simulink model "My_gfm_battery_sil_1"  (R2018b)
settings: Solver=ode23t  StartTime=0.0  StopTime=30  MaxStep=1e-4  RelTol=1e-3
PreLoadFcn:
  | modelDir = fileparts(get_param(bdroot,'FileName'));
  | 
  | load_system(fullfile(modelDir,'controls_element_lib.slx'));
  | load_system(fullfile(modelDir,'test_sequence_lib.slx'));
InitFcn:
  | close all;
  | clear all;
  | clc;
  | 
  | % frequency nominals
  | F_NOM = 60;
  | W_NOM = 2 * pi * F_NOM;
  | 
  | % base values relative to inverter
  | % --------------------------------
  | VLL_INV_NOM = 480;
  | P_INV_NOM = 1e6;
  | Q_INV_NOM = 0.5e6;
  | S_INV_NOM = sqrt(P_INV_NOM^2 + Q_INV_NOM^2);
  | 
  | I_INV_BASE = S_INV_NOM/(sqrt(3)*VLL_INV_NOM);
  | Z_INV_BASE = VLL_INV_NOM^2/S_INV_NOM;
  | L_INV_BASE = Z_INV_BASE / W_NOM;
  | C_INV_BASE = 1 / (Z_INV_BASE * W_NOM);
  | 
  | % nominal ratings for power system model
  | % --------------------------------------
  | INVERTER_COUNT = 100;
  | 
  | VLV_NOM = VLL_INV_NOM;
  | VMV_NOM = 35e3;
  | VHV_NOM = 230e3;
  | S_PLANT = INVERTER_COUNT * S_INV_NOM;
  | 
  | N_GSU = VHV_NOM/VMV_NOM;
  | N_MVT = VMV_NOM/VLV_NOM;
  | 
  | I_LV_BASE = S_PLANT/(sqrt(3)*VLV_NOM);
  | I_MV_BASE = S_PLANT/(sqrt(3)*VMV_NOM);
  | I_HV_BASE = S_PLANT/(sqrt(3)*VHV_NOM);
  | 
  | Z_LV_BASE = VLV_NOM^2/S_PLANT;
  | Z_MV_BASE = VMV_NOM^2/S_PLANT;
  | Z_HV_BASE = VHV_NOM^2/S_PLANT;
  | 
  | L_LV_BASE = Z_LV_BASE / W_NOM;
  | L_MV_BASE = Z_MV_BASE / W_NOM;
  | L_HV_BASE = Z_HV_BASE / W_NOM;
  | C_LV_BASE = 1 / (Z_LV_BASE * W_NOM);
  | C_MV_BASE = 1 / (Z_MV_BASE * W_NOM);
  | C_HV_BASE = 1 / (Z_HV_BASE * W_NOM);
undefined symbols (not defined in the file): j
libraries: simulink x38, test_sequence_lib x10, controls_element_lib x9
(part 1 of 5)
settings Model: SimulationMode=accelerator  Creator=HussamAlatrash  LastModifiedBy=ahhei
settings DataIOCC: ReturnWorkspaceOutputs=on
settings OptimizationCC: EfficientMapNaN2IntZero=off
settings DebuggingCC: UnconnectedInputMsg=none  UnconnectedOutputMsg=none  UnconnectedLineMsg=none
settings HardwareCC: TargetBitPerPointer=64  TargetBitPerSizeT=64  TargetBitPerPtrDiffT=64  TargetLongLongMode=on  TargetIntDivRoundTo=Zero  TargetEndianess=LittleEndian  TargetWordSize=64  TargetHWDeviceType=MATLAB Host  ProdEqTarget=off
settings ModelReferenceCC: EnableRefExpFcnMdlSchedulingChecks=off
settings CodeAppCC: MaxIdLength=128
settings GRTTargetCC: TargetLangStandard=C89/C90 (ANSI)  CombineOutputUpdateFcns=off  GRTInterface=on

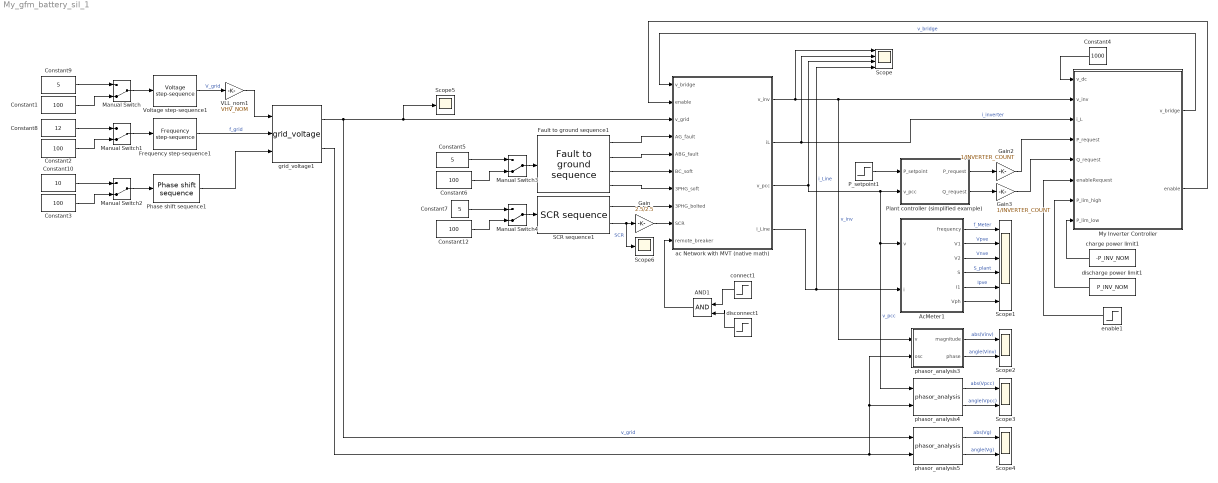
== system My_gfm_battery_sil_1 ==
  AND1 : Logic  IconShape=distinctive  AllPortsSameDT=off  OutDataTypeStr=boolean
  AcMeter1 : Subsystem  AncestorBlock=test_sequence_lib/AcMeter  mask{VllRated=VHV_NOM}
      mask prompts: VllRated "Rated line voltage"
  Constant{1..3,6,12} (5 alike) : Constant  Value=100
  Constant10 : Constant  Value=10
  Constant4 : Constant  Value=1000
  Constant5 : Constant  Value=5
  Constant7 : Constant  Value=5
  Constant8 : Constant  Value=12
  Constant9 : Constant  Value=5
  Fault to ground sequence1 : test_sequence_lib/Fault to ground sequence  SystemSampleTime=-1
  Frequency step-sequence1 : test_sequence_lib/Frequency step-sequence  SystemSampleTime=-1
  Gain : Gain  Gain=2.5/2.5
  Gain2 : Gain  Gain=1/INVERTER_COUNT
  Gain3 : Gain  Gain=1/INVERTER_COUNT
  Manual Switch{,1..4} (5 alike) : ManualSwitch  CurrentSetting=0
  "My Inverter Controller " : Subsystem
  P_setpoint1 : Step  Time=4  After=S_PLANT*0.9  SampleTime=0
  Phase shift sequence1 : test_sequence_lib/Phase shift sequence  SystemSampleTime=-1
  Plant controller (simplified example) : Subsystem  AncestorBlock=controls_element_lib/Battery plant controller
  SCR sequence1 : test_sequence_lib/SCR sequence  SystemSampleTime=-1
  Scope : Scope  NumInputPorts=4
  Scope1 : Scope  NumInputPorts=6
  Scope2 : Scope  NumInputPorts=2
  Scope3 : Scope  NumInputPorts=2
  Scope4 : Scope  NumInputPorts=2
  Scope5 : Scope
  Scope6 : Scope
  VLL_nom1 : Gain  Gain=VHV_NOM
  Voltage step-sequence1 : test_sequence_lib/Voltage step-sequence  SystemSampleTime=-1
  ac Network with MVT (native math) : Subsystem  AncestorBlock=test_sequence_lib/ac Network with MVT (native math)
  charge power limit1 : Constant  Value=-P_INV_NOM
  connect1 : Step  Time=0  SampleTime=0
  discharge power limit1 : Constant  Value=P_INV_NOM
  disconnect1 : Step  Time=100  Before=1  After=0  SampleTime=0
  enable1 : Step  Time=0.5  SampleTime=0
  grid_voltage1 : test_sequence_lib/grid_voltage  SystemSampleTime=-1
  phasor_analysis3 : Subsystem  AncestorBlock=test_sequence_lib/phasor_analysis
  phasor_analysis4 : test_sequence_lib/phasor_analysis  SystemSampleTime=-1
  phasor_analysis5 : test_sequence_lib/phasor_analysis  SystemSampleTime=-1
  wires:
  Voltage step-sequence1/1 -> VLL_nom1/1  "V_grid"
  Manual Switch/1 -> Voltage step-sequence1/1
  Fault to ground sequence1/2 -> ac Network with MVT (native math)/5(ABG_fault)
  AND1/1 -> ac Network with MVT (native math)/10(remote_breaker)
  Constant4/1 -> "My Inverter Controller "/1(v_dc)
  AcMeter1/3(V2) -> Scope1/3  "Vnve"
  discharge power limit1/1 -> "My Inverter Controller "/7(P_lim_high)
  Fault to ground sequence1/3 -> ac Network with MVT (native math)/6(BC_soft)
  AcMeter1/6(Vph) -> Scope1/6
  "My Inverter Controller "/1(v_bridge) -> ac Network with MVT (native math)/1(v_bridge)  "v_bridge"
  AcMeter1/2(V1) -> Scope1/2  "Vpve"
  Plant controller (simplified example)/1(P_request) -> Gain2/1
  ac Network with MVT (native math)/1(v_inv) -> phasor_analysis3/1(v), "My Inverter Controller "/2(v_inv), Scope/1  "v_inv"
  P_setpoint1/1 -> Plant controller (simplified example)/1(P_setpoint)
  phasor_analysis5/1 -> Scope4/1  "abs(Vg)"
  AcMeter1/5(I1) -> Scope1/5  "Ipve"
  Plant controller (simplified example)/2(Q_request) -> Gain3/1
  grid_voltage1/1 -> phasor_analysis5/1, Scope5/1, ac Network with MVT (native math)/3(v_grid)  "v_grid"
  SCR sequence1/1 -> ac Network with MVT (native math)/8(3PHG_bolted)
  phasor_analysis3/1(magnitude) -> Scope2/1  "abs(Vinv)"
  AcMeter1/4(S) -> Scope1/4  "S_plant"
  ac Network with MVT (native math)/4(i_Line) -> Scope/4, AcMeter1/2(i)  "i_Line"
  AcMeter1/1(frequency) -> Scope1/1  "f_Meter"
  VLL_nom1/1 -> grid_voltage1/1
  phasor_analysis3/2(phase) -> Scope2/2  "angle(Vinv)"
  SCR sequence1/2 -> Scope6/1, Gain/1  "SCR"
  ac Network with MVT (native math)/2(iL) -> "My Inverter Controller "/3(i_L), Scope/2  "i_inverter"
  disconnect1/1 -> AND1/2
  Fault to ground sequence1/4 -> ac Network with MVT (native math)/7(3PHG_soft)
  ac Network with MVT (native math)/3(v_pcc) -> Plant controller (simplified example)/2(v_pcc), phasor_analysis4/1, AcMeter1/1(v), Scope/3  "v_pcc"
  charge power limit1/1 -> "My Inverter Controller "/8(P_lim_low)
  "My Inverter Controller "/2(enable) -> ac Network with MVT (native math)/2(enable)
  Frequency step-sequence1/1 -> grid_voltage1/2  "f_grid"
  Fault to ground sequence1/1 -> ac Network with MVT (native math)/4(AG_fault)
  grid_voltage1/2 -> phasor_analysis4/2, phasor_analysis3/2(osc), phasor_analysis5/2
  phasor_analysis5/2 -> Scope4/2  "angle(Vg)"
  enable1/1 -> "My Inverter Controller "/6(enableRequest)
  connect1/1 -> AND1/1
  Constant9/1 -> Manual Switch/1
  Constant1/1 -> Manual Switch/2
  Constant2/1 -> Manual Switch1/2
  Manual Switch1/1 -> Frequency step-sequence1/1
  Constant8/1 -> Manual Switch1/1
  Manual Switch2/1 -> Phase shift sequence1/1
  Constant3/1 -> Manual Switch2/2
  Constant10/1 -> Manual Switch2/1
  Constant6/1 -> Manual Switch3/2
  Constant5/1 -> Manual Switch3/1
  Manual Switch3/1 -> Fault to ground sequence1/1
  Constant7/1 -> Manual Switch4/1
  Constant12/1 -> Manual Switch4/2
  Manual Switch4/1 -> SCR sequence1/1
  phasor_analysis4/1 -> Scope3/1  "abs(Vpcc)"
  phasor_analysis4/2 -> Scope3/2  "angle(Vpcc)"
  Phase shift sequence1/1 -> grid_voltage1/3
  Gain2/1 -> "My Inverter Controller "/4(P_request)
  Gain3/1 -> "My Inverter Controller "/5(Q_request)
  Gain/1 -> ac Network with MVT (native math)/9(SCR)

== system My_gfm_battery_sil_1/AcMeter1 ==
  v : Inport
  i : Inport  Port=2
  Conj : Math  Operator=conj  SaturateOnIntegerOverflow=on
  PLL_3ph : Subsystem
  Product : Product
  RMS calculator : Subsystem
  Scope : Scope  NumInputPorts=3
  Scope1 : Scope  NumInputPorts=4
  Sum of Elements : Sum  Commented=through  Inputs=+
  overVnom : Gain  Gain=1/VllRated
  phasor_analysis : Subsystem
  phasor_analysis1 : Subsystem  AncestorBlock=test_sequence_lib/AcMeter/phasor_analysis
  sqrt(3) : Gain  Gain=sqrt(3)
  sqrt(3)1 : Gain  Gain=sqrt(3)
  frequency : Outport  VectorParamsAs1DForOutWhenUnconnected=on
  V1 : Outport  Port=2  VectorParamsAs1DForOutWhenUnconnected=on
  V2 : Outport  Port=3  VectorParamsAs1DForOutWhenUnconnected=on
  S : Outport  Port=4  VectorParamsAs1DForOutWhenUnconnected=on
  I1 : Outport  Port=5  VectorParamsAs1DForOutWhenUnconnected=on
  Vph : Outport  Port=6  VectorParamsAs1DForOutWhenUnconnected=on
  wires:
  RMS calculator/1(out[3]) -> Vph/1
  PLL_3ph/2(osc[3]) -> phasor_analysis/2(osc), phasor_analysis1/2(osc)
  phasor_analysis/1(perPh) -> Scope/1
  Sum of Elements/1 -> Scope1/4, S/1  "S"
  v/1 -> RMS calculator/1(in[3]), phasor_analysis/1(in), overVnom/1
  PLL_3ph/1(freq) -> frequency/1
  overVnom/1 -> PLL_3ph/1(ref)
  Conj/1 -> Scope1/2, Product/2
  Product/1 -> Scope1/3, Sum of Elements/1
  phasor_analysis/2(pve) -> Scope/2, Scope1/1, Product/1, sqrt(3)/1  "Vpve_LN"
  phasor_analysis/3(nve) -> Scope/3, sqrt(3)1/1
  phasor_analysis1/2(pve) -> I1/1, Conj/1  "Ipve"
  sqrt(3)1/1 -> V2/1  "Vnve_LL"
  i/1 -> phasor_analysis1/1(in)
  sqrt(3)/1 -> V1/1  "Vpve_LL"

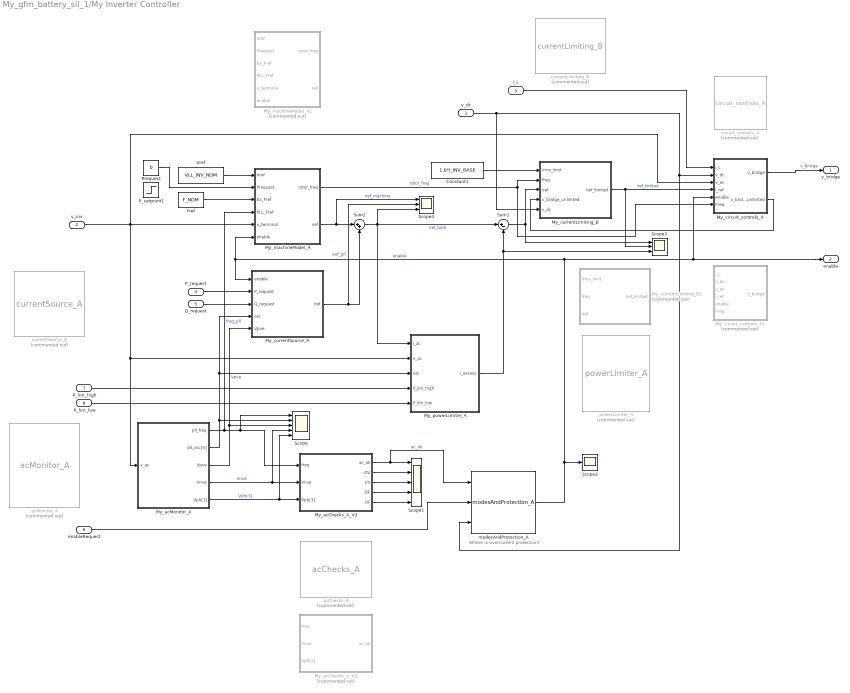
== system My_gfm_battery_sil_1/My Inverter Controller  ==
  note: Where is overcurrent protection?
  v_dc : Inport
  v_inv : Inport  Port=2
  i_L : Inport  Port=3
  P_request : Inport  Port=4
  Q_request : Inport  Port=5
  enableRequest : Inport  Port=6
  P_lim_high : Inport  Port=7
  P_lim_low : Inport  Port=8
  Constant1 : Constant  Value=1.6*I_INV_BASE
  Fref : Constant  Value=F_NOM
  My_acChecks_A_V2 : Subsystem  Commented=on  AncestorBlock=controls_element_lib/acChecks_A  mask{VllRated=VLL_INV_NOM, NominalFrequency=F_NOM, Ts=1e-3, Time1=2, Time2=0, VHi=1.15, VLo=0.85, FHi=62, FLo=58, VNeg=0.2, Time3=0, OV3=1.3, OV3_Time=0.02, OV3_en=1, OV2=1.25, OV2_Time=2, OV2_en=1, OV1=1.2, OV1_Time=20, OV1_en=1, UV1=0.81, UV1_Time=15, UV1_en=1, UV2=0.5, UV2_Time=5, UV2_en=1, UV3=0.2, UV3_Time=1, UV3_en=1, OF3=70, OF3_Time=0.2, OF3_en=1, OF2=65, OF2_Time=10, OF2_en=1, OF1=63, OF1_Time=30, OF1_en=1, UF1=56, UF1_Time=30, UF1_en=1, UF2=55, UF2_Time=10, UF2_en=1, UF3=50, UF3_Time=0.2, UF3_en=1}
      mask prompts: VllRated "Rated Line-to-Line Voltage (V)"; NominalFrequency "Nominal Line Frequency (Hz)"; Ts "Operating Sample Time (sec)"; Time1 "Connection Time (sec)"; Time2 "Connection Out-of-Condition Delay (sec)"; VHi "High Voltage Threshold (pu)"; VLo "Low Voltage Threshold (pu)"; FHi "High Frequency Threshold (Hz)"; FLo "Low Frequency Threshold (Hz)"; VNeg "Negative Sequence Voltage Threshold (pu)"; Time3 "Trip Out-of-Condition Delay (sec)"; OV3 "OV PickUp 3 (pu)"; OV3_Time "OV Time 3 (sec)"; OV3_en "OV Enable 3"; OV2 "OV PickUp 2 (pu)"; OV2_Time "OV Time 2 (sec)"; OV2_en "OV Enable 2"; OV1 "OV PickUp 1 (pu)"; OV1_Time "OV Time 1 (sec)"; OV1_en "OV Enable 1"; UV1 "UV PickUp 1 (pu)"; UV1_Time "UV Time 1 (sec)"; UV1_en "UV Enable 1"; UV2 "UV PickUp 2 (pu)"; UV2_Time "UV Time 2 (sec)"; UV2_en "UV Enable 2"; UV3 "UV PickUp 3 (pu)"; UV3_Time "UV Time 3 (sec)"; UV3_en "UV Enable 3"; OF3 "OF PickUp 3 (Hz)"; OF3_Time "OF Time 3 (pu)"; OF3_en "OF Enable 3"; OF2 "OF PickUp 2 (Hz)"; OF2_Time "OF Time 2 (pu)"; OF2_en "OF Enable 2"; OF1 "OF PickUp 1 (Hz)"; OF1_Time "OF Time 1 (pu)"; OF1_en "OF Enable 1"; UF1 "UF PickUp 1 (Hz)"; UF1_Time "UF Time 1 (sec)"; UF1_en "UF Enable 1"; UF2 "UF PickUp 2 (Hz)"; UF2_Time "UF Time 2 (sec)"; UF2_en "UF Enable 2"; UF3 "UF PickUp 3 (Hz)"; UF3_Time "UF Time 3 (sec)"; UF3_en "UF Enable 3"
      mask DialogControl DescGroupVar Prompt: ACChecks
      mask DialogControl DecsTextVar Prompt: Grid Checks for Connection and Tripping
      mask DialogControl ParameterGroupVar Prompt: General Parameters
      mask DialogControl Container11 Prompt: Connection Settings
      mask DialogControl Container20 Prompt: Thresholds
      mask DialogControl Container3 Prompt: Trip Settings
      mask DialogControl Container12 Prompt: General Parameters
      mask DialogControl Container15 Prompt: Over Voltage Settings
      mask DialogControl Container4 Prompt: Over Voltage
      mask DialogControl Container19 Prompt: Under Voltage Settings
      mask DialogControl Container7 Prompt: Under Voltage
      mask DialogControl Container17 Prompt: Over Frequency Settings
      mask DialogControl Container9 Prompt: Over Frequency
      mask DialogControl Container16 Prompt: Under Frequency Settings
      mask DialogControl Container10 Prompt: Under Frequency
  My_acChecks_A_V3 : Subsystem  AncestorBlock=controls_element_lib/acChecks_A  mask{VllRated=VLL_INV_NOM, NominalFrequency=F_NOM, Ts=1e-3, Time1=2, Time2=0, VHi=1.15, VLo=0.85, FHi=62, FLo=58, VNeg=0.2, Time3=0, OV3=1.3, OV3_Time=0.02, OV3_en=1, OV2=1.25, OV2_Time=2, OV2_en=1, OV1=1.2, OV1_Time=20, OV1_en=1, UV1=0.81, UV1_Time=15, UV1_en=1, UV2=0.5, UV2_Time=5, UV2_en=1, UV3=0.2, UV3_Time=1, UV3_en=1, OF3=70, OF3_Time=0.2, OF3_en=1, OF2=65, OF2_Time=10, OF2_en=1, OF1=63, OF1_Time=30, OF1_en=1, UF1=56, UF1_Time=30, UF1_en=1, UF2=55, UF2_Time=10, UF2_en=1, UF3=50, UF3_Time=0.2, UF3_en=1}
      mask prompts: VllRated "Rated Line-to-Line Voltage (V)"; NominalFrequency "Nominal Line Frequency (Hz)"; Ts "Operating Sample Time (sec)"; Time1 "Connection Time (sec)"; Time2 "Connection Out-of-Condition Delay (sec)"; VHi "High Voltage Threshold (pu)"; VLo "Low Voltage Threshold (pu)"; FHi "High Frequency Threshold (Hz)"; FLo "Low Frequency Threshold (Hz)"; VNeg "Negative Sequence Voltage Threshold (pu)"; Time3 "Trip Out-of-Condition Delay (sec)"; OV3 "OV PickUp 3 (pu)"; OV3_Time "OV Time 3 (sec)"; OV3_en "OV Enable 3"; OV2 "OV PickUp 2 (pu)"; OV2_Time "OV Time 2 (sec)"; OV2_en "OV Enable 2"; OV1 "OV PickUp 1 (pu)"; OV1_Time "OV Time 1 (sec)"; OV1_en "OV Enable 1"; UV1 "UV PickUp 1 (pu)"; UV1_Time "UV Time 1 (sec)"; UV1_en "UV Enable 1"; UV2 "UV PickUp 2 (pu)"; UV2_Time "UV Time 2 (sec)"; UV2_en "UV Enable 2"; UV3 "UV PickUp 3 (pu)"; UV3_Time "UV Time 3 (sec)"; UV3_en "UV Enable 3"; OF3 "OF PickUp 3 (Hz)"; OF3_Time "OF Time 3 (pu)"; OF3_en "OF Enable 3"; OF2 "OF PickUp 2 (Hz)"; OF2_Time "OF Time 2 (pu)"; OF2_en "OF Enable 2"; OF1 "OF PickUp 1 (Hz)"; OF1_Time "OF Time 1 (pu)"; OF1_en "OF Enable 1"; UF1 "UF PickUp 1 (Hz)"; UF1_Time "UF Time 1 (sec)"; UF1_en "UF Enable 1"; UF2 "UF PickUp 2 (Hz)"; UF2_Time "UF Time 2 (sec)"; UF2_en "UF Enable 2"; UF3 "UF PickUp 3 (Hz)"; UF3_Time "UF Time 3 (sec)"; UF3_en "UF Enable 3"
      mask DialogControl DescGroupVar Prompt: ACChecks
      mask DialogControl DecsTextVar Prompt: Grid Checks for Connection and Tripping
      mask DialogControl ParameterGroupVar Prompt: General Parameters
      mask DialogControl Container11 Prompt: Connection Settings
      mask DialogControl Container20 Prompt: Thresholds
      mask DialogControl Container3 Prompt: Trip Settings
      mask DialogControl Container12 Prompt: General Parameters
      mask DialogControl Container15 Prompt: Over Voltage Settings
      mask DialogControl Container4 Prompt: Over Voltage
      mask DialogControl Container19 Prompt: Under Voltage Settings
      mask DialogControl Container7 Prompt: Under Voltage
      mask DialogControl Container17 Prompt: Over Frequency Settings
      mask DialogControl Container9 Prompt: Over Frequency
      mask DialogControl Container16 Prompt: Under Frequency Settings
      mask DialogControl Container10 Prompt: Under Frequency
  My_acMonitor_A : Subsystem  AncestorBlock=controls_element_lib/acMonitor_A  mask{VllRated=VLL_INV_NOM, nominalFrequency=F_NOM}
      mask prompts: VllRated "Rated line-to-line voltage (V)"; nominalFrequency "Nominal line frequency (Hz)"
  My_circuit_controls_A : Subsystem  AncestorBlock=controls_element_lib/circuit_controls_A
  My_circuit_controls_A1 : Subsystem  Commented=on  AncestorBlock=controls_element_lib/circuit_controls_A
  My_currentLimiting_B : Subsystem  AncestorBlock=controls_element_lib/currentLimiting_B  mask{IRated=I_INV_BASE, peakSoftLimit=2.6, peakHardLimit=3.6}
      mask prompts: IRated "Rated current (A)"; peakSoftLimit "Soft peak limit (pu)"; peakHardLimit "Hard peak limit (pu)"
  My_currentLimiting_B1 : Subsystem  Commented=on  AncestorBlock=controls_element_lib/currentLimiting_B  mask{IRated=I_INV_BASE, peakSoftLimit=2.6, peakHardLimit=3.6}
      mask prompts: IRated "Rated current (A)"; peakSoftLimit "Soft peak limit (pu)"; peakHardLimit "Hard peak limit (pu)"
  My_currentSource_A : Subsystem  AncestorBlock=controls_element_lib/currentSource_A  mask{VllRated=VLL_INV_NOM, SRated=S_INV_NOM, nominalFrequency=F_NOM, Plimit=P_INV_NOM/S_INV_NOM, Qlimit=Q_INV_NOM/S_INV_NOM, CSOnline=1}
      mask prompts: VllRated "Rated line-to-line voltage (V)"; SRated "Rated power (VA)"; nominalFrequency "Nominal line frequency (Hz)"; Plimit "Real power request limit (pu)"; Qlimit "Reactive power request limit (pu)"; CSOnline "Current Source Online"
  My_machineModel_A : Subsystem  AncestorBlock=controls_element_lib/machineModel_A  mask{SRated=S_INV_NOM, VllRated=VLL_INV_NOM, nominalFrequency=F_NOM, MachOnline=1, inertialConstant=2.5, kDamper=2, tau_damp=0.3, Xs=0.3, rs=0.08, rn=0, wExciter=10, AVROnline=1, kqDroop=0, Xcomp=0, kp=5, ki=1, leak=10e-3, FreqRefSel=1, kDroop=1, wGoverner=1/0.3, kpSync=20, kpFastSync=1, wSync=2*pi*50, kpSyncFade=4, SyncFadeThres=0.2, tauMeas=0.02, tauBkSt=0.5}
      mask prompts: SRated "Rated power (VA)"; VllRated "Rated Voltage (Volts, line-to-line)"; nominalFrequency "Nominal frequency (Hz)"; MachOnline "Machine Online"; inertialConstant "Inertial constant (seconds)"; kDamper "Damper gain (pu/Hz)"; tau_damp "Damper time constant (sec)"; Xs "Stator reactance (pu)"; rs "Stator resistance (pu)"; rn "Neutral resistance (pu)"; wExciter "Exciter Bandwidth (rad)"; AVROnline "AVR Online"; kqDroop "QV Droop (pu v/ pu Q)"; Xcomp "Line drop compensation (pu)"; kp "Proportional gain"; ki "Integral gain"; leak "Leakage"; FreqRefSel "Frequency Reference Selector"; kDroop "Droop gain (pu/Hz)"; wGoverner "Governer Bandwidth (rad/s)"; kpSync "Synchronizer proportional gain (pu P / pu V)"; kpFastSync "Fast synchronizer gain (pu P / pu V)"; wSync "Synchronizer HPF Bandwidth(rad/s)"; kpSyncFade "Synchronizer fade gain (pu P/ puV)"; SyncFadeThres "Synchronizer fade threshold (pu)"; tauMeas "Measurements filters time constant (sec)"; tauBkSt "Black Start filter time constant (sec)"
      mask DialogControl DescGroupVar Prompt: Machine Model and Controls
      mask DialogControl ParameterGroupVar Prompt: Ratings
      mask DialogControl Container3 Prompt: Machine Parameters
      mask DialogControl Container4 Prompt: Mechanical Parameters
      mask DialogControl Container5 Prompt: Electrical Parameters
      mask DialogControl Container7 Prompt: AVR Parameters
      mask DialogControl Container6 Prompt: Governer Parameters
      mask DialogControl Container9 Prompt: Synchronizer Parameters
  My_machineModel_A1 : Subsystem  Commented=on  AncestorBlock=controls_element_lib/machineModel_A  mask{SRated=S_INV_NOM, VllRated=VLL_INV_NOM, nominalFrequency=F_NOM, inertialConstant=2.5, kDroop=1, kDamper=2, Xs=0.3, rs=0.08, Qlimit1=0.5, wExciter=10, FreqRefSel=1, MachOnline=0}
      mask prompts: SRated "Rated power (VA)"; VllRated "Rated Voltage (Volts, line-to-line)"; nominalFrequency "Nominal frequency (Hz)"; inertialConstant "Inertial constant (seconds)"; kDroop "Droop gain (pu/Hz)"; kDamper "Damper gain (pu/Hz)"; Xs "Stator reactance (pu)"; rs "Stator resistance (pu)"; Qlimit1 "Reactive power request limit (pu)"; wExciter "Exciter Bandwidth (rad)"; FreqRefSel "Frequency Reference Selector"; MachOnline "Machine Online"
      mask DialogControl DescGroupVar Prompt: Machine Model and Controls
  My_powerLimiter_A : Subsystem  AncestorBlock=controls_element_lib/powerLimiter_A  mask{VllRated=VLL_INV_NOM, nominalFrequency=F_NOM, wPowerLimiter=3}
      mask prompts: VllRated "Rated line-to-line voltage (V)"; nominalFrequency "Nominal line frequency (Hz)"; wPowerLimiter "Bandwidth (rad)"
  P_setpoint1 : Step  Time=4  After=S_PLANT*0.5  SampleTime=0
  Prequest : Constant  Value=0
  Scope : Scope  NumInputPorts=5
  Scope1 : Scope  NumInputPorts=5
  Scope2 : Scope
  Scope3 : Scope  NumInputPorts=3
  Scope4 : Scope  NumInputPorts=3
  Sum1 : Sum  Inputs=|+-
  Sum2 : Sum  Inputs=|++
  Vref : Constant  Value=VLL_INV_NOM
  acChecks_A : controls_element_lib/acChecks_A  Commented=on  VllRated=VLL_INV_NOM  nominalFrequency=F_NOM  tRequalify=2  T_CNTL=1e-3
  acMonitor_A : controls_element_lib/acMonitor_A  Commented=on  VllRated=VLL_INV_NOM  nominalFrequency=F_NOM
  circuit_controls_A : controls_element_lib/circuit_controls_A  Commented=on  SystemSampleTime=-1
  currentLimiting_B : controls_element_lib/currentLimiting_B  Commented=on  IRated=I_INV_BASE  peakSoftLimit=2.6  peakHardLimit=3.6
  currentSource_A : controls_element_lib/currentSource_A  Commented=on  VllRated=VLL_INV_NOM  SRated=S_INV_NOM  nominalFrequency=F_NOM  Plimit=P_INV_NOM/S_INV_NOM  Qlimit=Q_INV_NOM/S_INV_NOM
  modesAndProtection_A : controls_element_lib/modesAndProtection_A  dcOvervotlageThreshold=1800  dcUndervotlageThreshold=700  dcTripClearTimeout=0.2
  powerLimiter_A : controls_element_lib/powerLimiter_A  Commented=on  VllRated=VLL_INV_NOM  nominalFrequency=F_NOM  wPowerLimiter=3
  v_bridge : Outport  VectorParamsAs1DForOutWhenUnconnected=on
  enable : Outport  Port=2  VectorParamsAs1DForOutWhenUnconnected=on
  wires:
  Vref/1 -> My_machineModel_A/1(Vref)
  Prequest/1 -> My_machineModel_A/2(Prequest)
  My_machineModel_A/2(iref) -> Scope4/1, Sum2/1  "iref_machine"
  My_acMonitor_A/2(pll_osc[3]) -> Scope/2, My_currentSource_A/4(osc), My_powerLimiter_A/3(osc)
  My_currentLimiting_B/1(iref_limited) -> My_circuit_controls_A/4(i_ref), Scope3/2  "iref_limited"
  My_currentSource_A/1(iref) -> Sum2/2, Scope4/2  "iref_gfl"
  Sum2/1 -> Sum1/1, Scope4/3, My_powerLimiter_A/1(i_ac)  "iref_total"
  My_acMonitor_A/3(Vpve) -> My_currentSource_A/5(Vpve), Scope/3  "Vpve"
  Q_request/1 -> My_currentSource_A/3(Q_request)
  P_request/1 -> My_currentSource_A/2(P_request)
  enableRequest/1 -> modesAndProtection_A/2
  modesAndProtection_A/1 -> Scope2/1, My_machineModel_A/6(enable), My_currentSource_A/1(enable), My_circuit_controls_A/5(enable), enable/1  "enable"
  My_acMonitor_A/5(Vph[3]) -> My_acChecks_A_V3/3(Vph[3]), Scope/5  "Vph[3]"
  My_acChecks_A_V3/1(ac_ok) -> Scope1/1, modesAndProtection_A/1  "ac_ok"
  Constant1/1 -> My_currentLimiting_B/1(Irms_limit)
  My_acMonitor_A/1(pll_freq) -> My_machineModel_A/4(PLL_Fref), My_acChecks_A_V3/1(freq), Scope/1  "freq_pll"
  My_acMonitor_A/4(Vnve) -> My_acChecks_A_V3/2(Vnve), Scope/4  "Vnve"
  P_lim_low/1 -> My_powerLimiter_A/5(P_lim_low)
  P_lim_high/1 -> My_powerLimiter_A/4(P_lim_high)
  My_powerLimiter_A/1(i_excess) -> Sum1/2, Scope3/3
  Sum1/1 -> My_currentLimiting_B/3(iref), Scope3/1
  v_dc/1 -> My_circuit_controls_A/2(v_dc), modesAndProtection_A/3, My_currentLimiting_B/5(v_dc)
  My_circuit_controls_A/1(v_bridge) -> v_bridge/1  "v_bridge"
  My_machineModel_A/1(rotor_freq) -> My_circuit_controls_A/6(Freq), My_currentLimiting_B/2(freq)  "rotor_freq"
  i_L/1 -> My_circuit_controls_A/1(i_L)
  v_inv/1 -> My_machineModel_A/5(v_terminal), My_circuit_controls_A/3(v_ac), My_acMonitor_A/1(v_ac), My_powerLimiter_A/2(v_ac)
  Fref/1 -> My_machineModel_A/3(Ex_Fref)
  My_acChecks_A_V3/2(OV) -> Scope1/2
  My_acChecks_A_V3/3(UV) -> Scope1/3
  My_acChecks_A_V3/4(OF) -> Scope1/4
  My_acChecks_A_V3/5(UF) -> Scope1/5
  My_circuit_controls_A/2(v_bridge_unlimted) -> My_currentLimiting_B/4(v_bridge_unlimted)

== system My_gfm_battery_sil_1/Plant controller (simplified example) ==
  P_setpoint : Inport
  v_pcc : Inport  Port=2
  Gain : Gain  Gain=-1
  Gain1 : Gain  Gain=S_PLANT
  Gain2 : Gain  Gain=S_PLANT
  Gain4 : Gain  Gain=1/VHV_NOM
  LVRT_foldback : Subsystem
  Meter : Subsystem
  Saturation : Saturate  UpperLimit=0.9*S_PLANT  LowerLimit=-0.9*S_PLANT
  Saturation Dynamic : simulink/Discontinuities/Saturation Dynamic  OutMin=[]  OutMax=[]  OutDataTypeStr=Inherit: Same as second input  OutDataType=fixdt(1, 16)  OutScaling=2^-10  DoSatur=off
  Scope : Scope  NumInputPorts=5
  VoltVAr : Subsystem
  P_request : Outport  VectorParamsAs1DForOutWhenUnconnected=on
  Q_request : Outport  Port=2  VectorParamsAs1DForOutWhenUnconnected=on
  wires:
  Gain/1 -> Saturation Dynamic/3
  Saturation Dynamic/1 -> Scope/1, P_request/1  "P_request"
  LVRT_foldback/1(limit_pu) -> Scope/2, Gain2/1  "spinout_limit_Vpcc"
  Gain2/1 -> Saturation Dynamic/1, Gain/1
  Saturation/1 -> Saturation Dynamic/2
  Gain4/1 -> Scope/5, Meter/1(v)
  P_setpoint/1 -> Saturation/1
  v_pcc/1 -> Gain4/1
  Gain1/1 -> Q_request/1  "Q_request"
  Meter/1(Vpve) -> Scope/4, VoltVAr/1(Vpve_pu), LVRT_foldback/1(Vpve_pu)  "V_pu_plant"
  VoltVAr/1(Q) -> Gain1/1, Scope/3

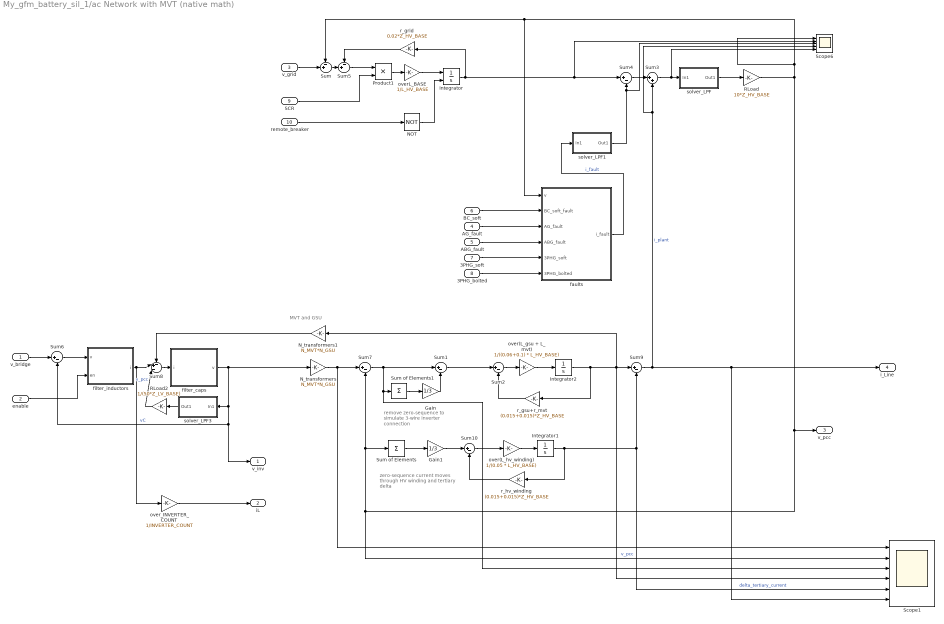
== system My_gfm_battery_sil_1/ac Network with MVT (native math) ==
  note: zero-sequence current moves through HV winding and tertiary delta
  note: remove zero-sequence to simulate 3-wire inverter connection
  note: MVT and GSU
  v_bridge : Inport
  enable : Inport  Port=2
  v_grid : Inport  Port=3
  AG_fault : Inport  Port=4
  ABG_fault : Inport  Port=5
  BC_soft : Inport  Port=6
  3PHG_soft : Inport  Port=7
  3PHG_bolted : Inport  Port=8
  SCR : Inport  Port=9
  remote_breaker : Inport  Port=10
  Gain : Gain  Gain=1/3
  Gain1 : Gain  Gain=1/3
  Integrator : Integrator  ExternalReset=level
  Integrator1 : Integrator
  Integrator2 : Integrator
  NOT : Logic  Operator=NOT  IconShape=distinctive  AllPortsSameDT=off  OutDataTypeStr=boolean
  N_transformers : Gain  Gain=N_MVT*N_GSU
  N_transformers1 : Gain  Gain=N_MVT*N_GSU
  Product1 : Product
  RLoad : Gain  Gain=10*Z_HV_BASE
  RLoad2 : Gain  Gain=1/(50*Z_LV_BASE)
  Scope1 : Scope  NumInputPorts=6
  Scope6 : Scope  NumInputPorts=5
  Sum : Sum  Inputs=-+|
  Sum of Elements : Sum  Inputs=+
  Sum of Elements1 : Sum  Inputs=+
  Sum{1..2,4,6..7,9..10} (7 alike) : Sum  Inputs=|+-
  Sum3 : Sum  Inputs=|++
  Sum5 : Sum  Inputs=-+|
  Sum8 : Sum  Inputs=-+-|
  faults : Subsystem
  filter_caps : Subsystem
  filter_inductors : Subsystem
  over(L_gsu + L_mvt) : Gain  Gain=1/((0.06+0.1) * L_HV_BASE)
  over(L_hv_winding) : Gain  Gain=1/(0.05 * L_HV_BASE)
  overL_BASE : Gain  Gain=1/L_HV_BASE
  over_INVERTER_COUNT : Gain  Gain=1/INVERTER_COUNT
  r_grid : Gain  Gain=0.02*Z_HV_BASE
  r_gsu+r_mvt : Gain  Gain=(0.015+0.015)*Z_HV_BASE
  r_hv_winding : Gain  Gain=(0.015+0.015)*Z_HV_BASE
  solver_LPF : Subsystem
  solver_LPF1 : Subsystem
  solver_LPF3 : Subsystem
  v_inv : Outport  VectorParamsAs1DForOutWhenUnconnected=on
  iL : Outport  Port=2  VectorParamsAs1DForOutWhenUnconnected=on
  v_pcc : Outport  Port=3  VectorParamsAs1DForOutWhenUnconnected=on
  i_Line : Outport  Port=4  VectorParamsAs1DForOutWhenUnconnected=on
  wires:
  AG_fault/1 -> faults/3(AG_fault)
  ABG_fault/1 -> faults/4(ABG_fault)
  BC_soft/1 -> faults/2(BC_soft_fault)
  Gain1/1 -> Sum10/1
  Sum of Elements/1 -> Gain1/1
  Sum10/1 -> over(L_hv_winding)/1
  r_hv_winding/1 -> Sum10/2
  Integrator1/1 -> r_hv_winding/1, Scope1/5, Sum9/2  "delta_tertiary_current"
  over(L_hv_winding)/1 -> Integrator1/1
  Sum9/1 -> Scope1/6, i_Line/1, Scope6/4, Sum3/2  "i_plant"
  N_transformers1/1 -> Sum8/1
  N_transformers/1 -> Scope1/1, Sum7/1
  over_INVERTER_COUNT/1 -> iL/1
  filter_caps/1(v) -> N_transformers/1, solver_LPF3/1(In1), Sum6/2, v_inv/1  "vC"
  Sum8/1 -> filter_caps/1(i)
  filter_inductors/1(i) -> over_INVERTER_COUNT/1, Sum8/2
  enable/1 -> filter_inductors/2(en)
  Sum6/1 -> filter_inductors/1(v)
  r_gsu+r_mvt/1 -> Sum2/2
  Sum1/1 -> Sum2/1
  Gain/1 -> Sum1/2
  Sum of Elements1/1 -> Gain/1
  Sum2/1 -> over(L_gsu + L_mvt)/1
  Sum7/1 -> Sum1/1, Scope1/3, Sum of Elements1/1
  over(L_gsu + L_mvt)/1 -> Integrator2/1
  solver_LPF/1(Out1) -> RLoad/1
  remote_breaker/1 -> NOT/1
  overL_BASE/1 -> Integrator/1
  Integrator/1 -> Scope6/2, Sum4/1, r_grid/1
  solver_LPF1/1(Out1) -> Scope6/3, Sum4/2
  RLoad/1 -> Sum of Elements/1, Sum7/2, Scope1/2, v_pcc/1, Sum/1, faults/1(v), Scope6/1  "v_pcc"
  faults/1(i_fault) -> solver_LPF1/1(In1)  "i_fault"
  3PHG_bolted/1 -> faults/6(3PHG_bolted)
  v_bridge/1 -> Sum6/1
  Product1/1 -> overL_BASE/1
  SCR/1 -> Product1/2
  r_grid/1 -> Sum5/1
  Sum3/1 -> Scope6/5, solver_LPF/1(In1)
  NOT/1 -> Integrator/2
  Sum4/1 -> Sum3/1
  v_grid/1 -> Sum/2
  Sum5/1 -> Product1/1
  Sum/1 -> Sum5/2
  Integrator2/1 -> Scope1/4, Sum9/1, N_transformers1/1, r_gsu+r_mvt/1
  3PHG_soft/1 -> faults/5(3PHG_soft)
  solver_LPF3/1(Out1) -> RLoad2/1
  RLoad2/1 -> Sum8/3  "v_pcc"

== system My_gfm_battery_sil_1/phasor_analysis3 ==
  v : Inport
  osc : Inport  Port=2
  Complex to Magnitude-Angle : ComplexToMagnitudeAngle
  Complex to Real-Imag : ComplexToRealImag
  Conj : Math  Operator=conj  SaturateOnIntegerOverflow=on
  Gain : Gain  Gain=sqrt(2)
  Gain1 : Gain  Gain=1/3
  Gain2 : Gain  Gain=sqrt(3)
  Product3 : Product
  Real-Imag to Complex : RealImagToComplex
  Scope : Scope  NumInputPorts=4
  Sum of Elements1 : Sum  Inputs=+
  Transfer Fcn : TransferFcn  Denominator=[0.01 1]
  Transfer Fcn1 : TransferFcn  Denominator=[0.01 1]
  magnitude : Outport  VectorParamsAs1DForOutWhenUnconnected=on
  phase : Outport  Port=2  VectorParamsAs1DForOutWhenUnconnected=on
  wires:
  Complex to Magnitude-Angle/2 -> phase/1
  Complex to Magnitude-Angle/1 -> magnitude/1
  Gain2/1 -> Complex to Magnitude-Angle/1
  Gain1/1 -> Complex to Real-Imag/1
  Gain/1 -> Scope/2, Product3/2
  Real-Imag to Complex/1 -> Gain2/1
  Conj/1 -> Gain/1
  osc/1 -> Conj/1
  Complex to Real-Imag/1 -> Transfer Fcn/1
  v/1 -> Scope/1, Product3/1
  Complex to Real-Imag/2 -> Transfer Fcn1/1
  Product3/1 -> Scope/3, Sum of Elements1/1
  Transfer Fcn/1 -> Real-Imag to Complex/1
  Sum of Elements1/1 -> Scope/4, Gain1/1
  Transfer Fcn1/1 -> Real-Imag to Complex/2

== system My_gfm_battery_sil_1/AcMeter1/PLL_3ph ==
  ref : Inport
  Complex to Real-Imag : ComplexToRealImag
  Conj : Math  Operator=conj  SaturateOnIntegerOverflow=on
  Constant : Constant  Value=120
  Gain1 : Gain  Gain=1.5
  Gain2 : Gain  Gain=4.5
  Gain3 : Gain  Gain=10e-3
  Integrator : Integrator  LimitOutput=on  UpperSaturationLimit=5  LowerSaturationLimit=-5
  Product : Product
  SOGI : Subsystem  AncestorBlock=controls_module_lib/dcVoltageRegulator_A/SOGI
  Saturation : Saturate  UpperLimit=5  LowerLimit=-5
  Sum : Sum  Inputs=+++
  Sum of Elements : Sum  Inputs=+
  Sum1 : Sum  Inputs=|+-
  Transfer Fcn : TransferFcn  Denominator=[0.02 1]
  f_nom : Constant  Value=60
  oscillator_3ph : Subsystem
  freq : Outport  VectorParamsAs1DForOutWhenUnconnected=on
  osc[3] : Outport  Port=2  VectorParamsAs1DForOutWhenUnconnected=on
  wires:
  Gain1/1 -> Saturation/1
  Conj/1 -> Complex to Real-Imag/1
  ref/1 -> Product/1
  Integrator/1 -> Sum/3, Gain3/1
  Sum1/1 -> Integrator/1
  Complex to Real-Imag/2 -> Product/2
  Gain2/1 -> Sum1/1
  oscillator_3ph/1(osc[3]) -> osc[3]/1, Conj/1
  Sum/1 -> oscillator_3ph/1(f), freq/1  "freq"
  Product/1 -> Sum of Elements/1
  Saturation/1 -> Sum/2
  SOGI/1(notch) -> Gain2/1, Gain1/1  "phase_error"
  Sum of Elements/1 -> Transfer Fcn/1
  Gain3/1 -> Sum1/2
  f_nom/1 -> Sum/1
  Transfer Fcn/1 -> SOGI/1(in)  "phase_error"
  Constant/1 -> SOGI/2(fnom)

== system My_gfm_battery_sil_1/AcMeter1/RMS calculator ==
  in[3] : Inport
  Gain : Gain  Gain=20
  Integrator : Integrator
  Square : Math  Operator=square  SaturateOnIntegerOverflow=on
  Square Root : Sqrt  SaturateOnIntegerOverflow=on
  Sum : Sum  Inputs=|+-
  out[3] : Outport  VectorParamsAs1DForOutWhenUnconnected=on
  wires:
  in[3]/1 -> Square/1
  Square/1 -> Sum/1
  Gain/1 -> Integrator/1
  Square Root/1 -> out[3]/1  "Vph_rms"
  Sum/1 -> Gain/1
  Integrator/1 -> Square Root/1, Sum/2

== system My_gfm_battery_sil_1/AcMeter1/phasor_analysis ==
  in : Inport
  osc : Inport  Port=2
  Conj : Math  Operator=conj  SaturateOnIntegerOverflow=on
  Conj1 : Math  Operator=conj  SaturateOnIntegerOverflow=on
  Demux : Demux  Outputs=3
  Gain1 : Gain  Gain=1/3
  Gain3 : Gain  Gain=1/3
  Mux : Mux  Inputs=3
  Product1 : Product
  Product3 : Product
  Scope : Scope  NumInputPorts=5
  Sum of Elements1 : Sum  Inputs=+
  Sum of Elements2 : Sum  Inputs=+
  complex_LPF1 : Subsystem  mask{wLPF=50}
      mask prompts: wLPF "Bandwidth (rad/sec)"
  complex_LPF2 : test_sequence_lib/AcMeter/phasor_analysis/complex_LPF1  wLPF=50
  sqrt(2) : Gain  Gain=sqrt(2)
  sqrt(2)1 : Gain  Gain=sqrt(2)
  perPh : Outport  VectorParamsAs1DForOutWhenUnconnected=on
  pve : Outport  Port=2  VectorParamsAs1DForOutWhenUnconnected=on
  nve : Outport  Port=3  VectorParamsAs1DForOutWhenUnconnected=on
  wires:
  complex_LPF2/1 -> Sum of Elements2/1
  Product1/1 -> complex_LPF2/1
  complex_LPF1/1(1) -> Scope/4, perPh/1
  Product3/1 -> Sum of Elements1/1, Scope/3, complex_LPF1/1(In1)
  Sum of Elements1/1 -> Scope/5, Gain1/1
  in/1 -> Scope/1, Product3/1, Product1/1
  osc/1 -> Demux/1, Conj/1
  Conj/1 -> sqrt(2)/1
  sqrt(2)/1 -> Scope/2, Product3/2
  Gain1/1 -> pve/1
  Demux/1 -> Mux/1
  Demux/2 -> Mux/3
  Demux/3 -> Mux/2
  Mux/1 -> Conj1/1
  Conj1/1 -> sqrt(2)1/1
  sqrt(2)1/1 -> Product1/2
  Sum of Elements2/1 -> Gain3/1
  Gain3/1 -> nve/1

== system My_gfm_battery_sil_1/AcMeter1/phasor_analysis1 ==
  in : Inport
  osc : Inport  Port=2
  Conj : Math  Operator=conj  SaturateOnIntegerOverflow=on
  Conj1 : Math  Operator=conj  SaturateOnIntegerOverflow=on
  Demux : Demux  Outputs=3
  Gain1 : Gain  Gain=1/3
  Gain3 : Gain  Gain=1/3
  Mux : Mux  Inputs=3
  Product1 : Product
  Product3 : Product
  Sum of Elements1 : Sum  Inputs=+
  Sum of Elements2 : Sum  Inputs=+
  complex_LPF1 : Subsystem  Commented=through  mask{wLPF=50}
      mask prompts: wLPF "Bandwidth (rad/sec)"
  complex_LPF2 : test_sequence_lib/AcMeter/phasor_analysis/complex_LPF1  wLPF=50
  sqrt(2) : Gain  Gain=sqrt(2)
  sqrt(2)1 : Gain  Gain=sqrt(2)
  perPh : Outport  VectorParamsAs1DForOutWhenUnconnected=on
  pve : Outport  Port=2  VectorParamsAs1DForOutWhenUnconnected=on
  nve : Outport  Port=3  VectorParamsAs1DForOutWhenUnconnected=on
  wires:
  complex_LPF2/1 -> Sum of Elements2/1
  Product1/1 -> complex_LPF2/1
  complex_LPF1/1(1) -> perPh/1, Sum of Elements1/1
  Product3/1 -> complex_LPF1/1(In1)
  Sum of Elements1/1 -> Gain1/1
  in/1 -> Product3/1, Product1/1
  osc/1 -> Demux/1, Conj/1
  Conj/1 -> sqrt(2)/1
  sqrt(2)/1 -> Product3/2
  Gain1/1 -> pve/1
  Demux/1 -> Mux/1
  Demux/2 -> Mux/3
  Demux/3 -> Mux/2
  Mux/1 -> Conj1/1
  Conj1/1 -> sqrt(2)1/1
  sqrt(2)1/1 -> Product1/2
  Sum of Elements2/1 -> Gain3/1
  Gain3/1 -> nve/1

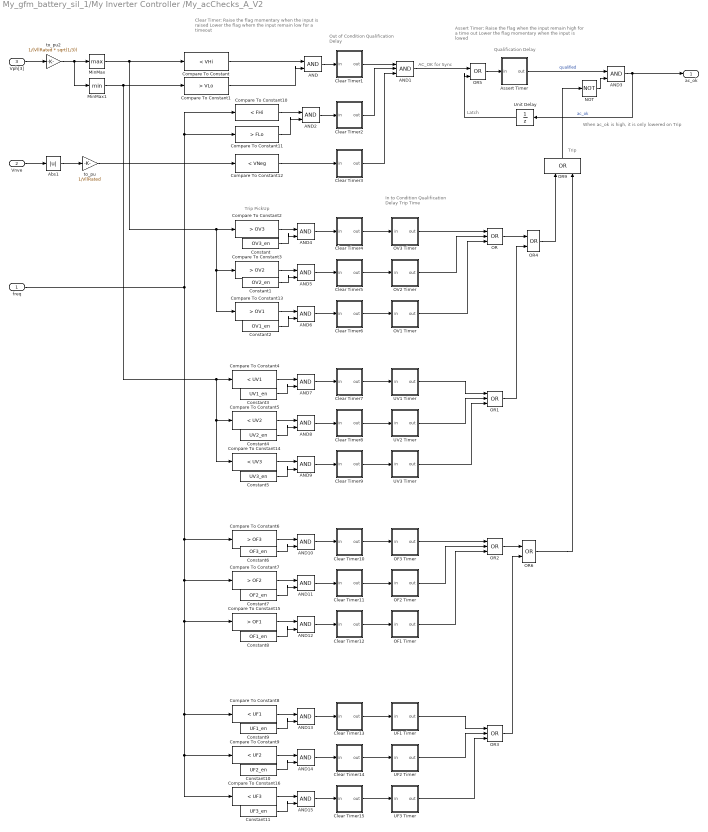
== system My_gfm_battery_sil_1/My Inverter Controller /My_acChecks_A_V2 ==
  note: Trip
  note: Clear Timer:
      | Raise the flag momentary when the input is raised
      | Lower the flag whern the input remain low for a timeout
  note: AC_OK for Sync
  note: Assert Timer:
      | Raise the flag when the input remain high for a time out
      | Lower the flag momentary when the input is lowed
  note: Latch
  note: Qualification Delay
  note: When ac_ok is high, it is only lowered on Trip
  note: Out of Condition
      | Qualification Delay
  note: In to Condition
      | Qualification Delay
      | Trip Time
  note: Trip PickUp
  freq : Inport
  Vnve : Inport  Port=2
  Vph[3] : Inport  Port=3
  AND{,2..15} (15 alike) : Logic  IconShape=distinctive  AllPortsSameDT=off  OutDataTypeStr=boolean
  AND1 : Logic  Inputs=3  IconShape=distinctive  AllPortsSameDT=off  OutDataTypeStr=boolean
  Abs1 : Abs
  Assert Timer : Subsystem  mask{T_STEP=Ts, TIMEOUT=Time1}
      mask prompts: T_STEP "Time step"
  Clear Timer1 : Subsystem  mask{T_STEP=Ts, TIMEOUT=Time2, TIMER_INIT=0}
      mask prompts: T_STEP "Time step"; TIMER_INIT "Timer initial value"
  Clear Timer10 : Subsystem  mask{T_STEP=Ts, TIMEOUT=Time3, TIMER_INIT=0}
      mask prompts: T_STEP "Time step"; TIMER_INIT "Timer initial value"
  Clear Timer11 : Subsystem  mask{T_STEP=Ts, TIMEOUT=Time3, TIMER_INIT=0}
      mask prompts: T_STEP "Time step"; TIMER_INIT "Timer initial value"
  Clear Timer12 : Subsystem  mask{T_STEP=Ts, TIMEOUT=Time3, TIMER_INIT=0}
      mask prompts: T_STEP "Time step"; TIMER_INIT "Timer initial value"
  Clear Timer13 : Subsystem  mask{T_STEP=Ts, TIMEOUT=Time3, TIMER_INIT=0}
      mask prompts: T_STEP "Time step"; TIMER_INIT "Timer initial value"
  Clear Timer14 : Subsystem  mask{T_STEP=Ts, TIMEOUT=Time3, TIMER_INIT=0}
      mask prompts: T_STEP "Time step"; TIMER_INIT "Timer initial value"
  Clear Timer15 : Subsystem  mask{T_STEP=Ts, TIMEOUT=Time3, TIMER_INIT=0}
      mask prompts: T_STEP "Time step"; TIMER_INIT "Timer initial value"
  Clear Timer2 : Subsystem  mask{T_STEP=Ts, TIMEOUT=Time2, TIMER_INIT=0}
      mask prompts: T_STEP "Time step"; TIMER_INIT "Timer initial value"
  Clear Timer3 : Subsystem  mask{T_STEP=Ts, TIMEOUT=Time2, TIMER_INIT=0}
      mask prompts: T_STEP "Time step"; TIMER_INIT "Timer initial value"
  Clear Timer4 : Subsystem  mask{T_STEP=Ts, TIMEOUT=Time3, TIMER_INIT=0}
      mask prompts: T_STEP "Time step"; TIMER_INIT "Timer initial value"
  Clear Timer5 : Subsystem  mask{T_STEP=Ts, TIMEOUT=Time3, TIMER_INIT=0}
      mask prompts: T_STEP "Time step"; TIMER_INIT "Timer initial value"
  Clear Timer6 : Subsystem  mask{T_STEP=Ts, TIMEOUT=Time3, TIMER_INIT=0}
      mask prompts: T_STEP "Time step"; TIMER_INIT "Timer initial value"
  Clear Timer7 : Subsystem  mask{T_STEP=Ts, TIMEOUT=Time3, TIMER_INIT=0}
      mask prompts: T_STEP "Time step"; TIMER_INIT "Timer initial value"
  Clear Timer8 : Subsystem  mask{T_STEP=Ts, TIMEOUT=Time3, TIMER_INIT=0}
      mask prompts: T_STEP "Time step"; TIMER_INIT "Timer initial value"
  Clear Timer9 : Subsystem  mask{T_STEP=Ts, TIMEOUT=Time3, TIMER_INIT=0}
      mask prompts: T_STEP "Time step"; TIMER_INIT "Timer initial value"
  Compare To Constant : simulink/Logic and Bit Operations/Compare To Constant  relop=<  const=VHi  OutDataTypeStr=boolean
  Compare To Constant1 : simulink/Logic and Bit Operations/Compare To Constant  relop=>  const=VLo  OutDataTypeStr=boolean
  Compare To Constant10 : simulink/Logic and Bit Operations/Compare To Constant  relop=<  const=FHi  OutDataTypeStr=boolean
  Compare To Constant11 : simulink/Logic and Bit Operations/Compare To Constant  relop=>  const=FLo  OutDataTypeStr=boolean
  Compare To Constant12 : simulink/Logic and Bit Operations/Compare To Constant  relop=<  const=VNeg  OutDataTypeStr=boolean
  Compare To Constant13 : simulink/Logic and Bit Operations/Compare To Constant  relop=>  const=OV1  OutDataTypeStr=boolean
  Compare To Constant14 : simulink/Logic and Bit Operations/Compare To Constant  relop=<  const=UV3  OutDataTypeStr=boolean
  Compare To Constant15 : simulink/Logic and Bit Operations/Compare To Constant  relop=>  const=OF1  OutDataTypeStr=boolean
  Compare To Constant16 : simulink/Logic and Bit Operations/Compare To Constant  relop=<  const=UF3  OutDataTypeStr=boolean
  Compare To Constant2 : simulink/Logic and Bit Operations/Compare To Constant  relop=>  const=OV3  OutDataTypeStr=boolean
  Compare To Constant3 : simulink/Logic and Bit Operations/Compare To Constant  relop=>  const=OV2  OutDataTypeStr=boolean
  Compare To Constant4 : simulink/Logic and Bit Operations/Compare To Constant  relop=<  const=UV1  OutDataTypeStr=boolean
  Compare To Constant5 : simulink/Logic and Bit Operations/Compare To Constant  relop=<  const=UV2  OutDataTypeStr=boolean
  Compare To Constant6 : simulink/Logic and Bit Operations/Compare To Constant  relop=>  const=OF3  OutDataTypeStr=boolean
  Compare To Constant7 : simulink/Logic and Bit Operations/Compare To Constant  relop=>  const=OF2  OutDataTypeStr=boolean
  Compare To Constant8 : simulink/Logic and Bit Operations/Compare To Constant  relop=<  const=UF1  OutDataTypeStr=boolean
  Compare To Constant9 : simulink/Logic and Bit Operations/Compare To Constant  relop=<  const=UF2  OutDataTypeStr=boolean
  Constant : Constant  Value=OV3_en
  Constant1 : Constant  Value=OV2_en
  Constant10 : Constant  Value=UF2_en
  Constant11 : Constant  Value=UF3_en
  Constant2 : Constant  Value=OV1_en
  Constant3 : Constant  Value=UV1_en
  Constant4 : Constant  Value=UV2_en
  Constant5 : Constant  Value=UV3_en
  Constant6 : Constant  Value=OF3_en
  Constant7 : Constant  Value=OF2_en
  Constant8 : Constant  Value=OF1_en
  Constant9 : Constant  Value=UF1_en
  MinMax : MinMax  Function=max
  MinMax1 : MinMax
  NOT : Logic  Operator=NOT  IconShape=distinctive  AllPortsSameDT=off  OutDataTypeStr=boolean
  OF1 Timer : Subsystem  mask{T_STEP=Ts, TIMEOUT=OF1_Time}
      mask prompts: T_STEP "Time step"
  OF2 Timer : Subsystem  mask{T_STEP=Ts, TIMEOUT=OF2_Time}
      mask prompts: T_STEP "Time step"
  OF3 Timer : Subsystem  mask{T_STEP=Ts, TIMEOUT=OF3_Time}
      mask prompts: T_STEP "Time step"
  OR{,1..3} (4 alike) : Logic  Operator=OR  Inputs=3  IconShape=distinctive  AllPortsSameDT=off  OutDataTypeStr=boolean
  OR{4..6,9} (4 alike) : Logic  Operator=OR  IconShape=distinctive  AllPortsSameDT=off  OutDataTypeStr=boolean
  OV1 Timer : Subsystem  mask{T_STEP=Ts, TIMEOUT=OV1_Time}
      mask prompts: T_STEP "Time step"
  OV2 Timer : Subsystem  mask{T_STEP=Ts, TIMEOUT=OV2_Time}
      mask prompts: T_STEP "Time step"
  OV3 Timer : Subsystem  mask{T_STEP=Ts, TIMEOUT=OV3_Time}
      mask prompts: T_STEP "Time step"
  UF1 Timer : Subsystem  mask{T_STEP=Ts, TIMEOUT=UF1_Time}
      mask prompts: T_STEP "Time step"
  UF2 Timer : Subsystem  mask{T_STEP=Ts, TIMEOUT=UF2_Time}
      mask prompts: T_STEP "Time step"
  UF3 Timer : Subsystem  mask{T_STEP=Ts, TIMEOUT=UF3_Time}
      mask prompts: T_STEP "Time step"
  UV1 Timer : Subsystem  mask{T_STEP=Ts, TIMEOUT=UV1_Time}
      mask prompts: T_STEP "Time step"
  UV2 Timer : Subsystem  mask{T_STEP=Ts, TIMEOUT=UV2_Time}
      mask prompts: T_STEP "Time step"
  UV3 Timer : Subsystem  mask{T_STEP=Ts, TIMEOUT=UV3_Time}
      mask prompts: T_STEP "Time step"
  Unit Delay : UnitDelay  SampleTime=Ts
  to_pu : Gain  Gain=1/VllRated
  to_pu2 : Gain  Gain=1/(VllRated * sqrt(1/3))
  ac_ok : Outport  VectorParamsAs1DForOutWhenUnconnected=on
  wires:
  Vph[3]/1 -> to_pu2/1
  OR4/1 -> OR9/1
  OR9/1 -> NOT/1
  to_pu/1 -> Compare To Constant12/1
  MinMax/1 -> Compare To Constant13/1, Compare To Constant3/1, Compare To Constant2/1, Compare To Constant/1
  Abs1/1 -> to_pu/1
  Unit Delay/1 -> OR5/2
  OV3 Timer/1(out) -> OR/1
  Compare To Constant12/1 -> Clear Timer3/1(in)
  Clear Timer3/1(out) -> AND1/3
  Assert Timer/1(out) -> AND3/1  "qualified"
  UV2 Timer/1(out) -> OR1/2
  OF3 Timer/1(out) -> OR2/1
  Clear Timer10/1(out) -> OF3 Timer/1(in)
  Compare To Constant6/1 -> AND10/1
  Clear Timer11/1(out) -> OF2 Timer/1(in)
  Clear Timer4/1(out) -> OV3 Timer/1(in)
  UF1 Timer/1(out) -> OR3/1
  UF2 Timer/1(out) -> OR3/2
  Vnve/1 -> Abs1/1
  NOT/1 -> AND3/2
  UV1 Timer/1(out) -> OR1/1
  AND2/1 -> Clear Timer2/1(in)
  Compare To Constant11/1 -> AND2/2
  OF2 Timer/1(out) -> OR2/2
  Clear Timer7/1(out) -> UV1 Timer/1(in)
  OR1/1 -> OR4/2
  Clear Timer13/1(out) -> UF1 Timer/1(in)
  Compare To Constant7/1 -> AND11/1
  Clear Timer2/1(out) -> AND1/2
  Clear Timer14/1(out) -> UF2 Timer/1(in)
  Clear Timer5/1(out) -> OV2 Timer/1(in)
  freq/1 -> Compare To Constant11/1, Compare To Constant10/1, Compare To Constant8/1, Compare To Constant16/1, Compare To Constant9/1, Compare To Constant15/1, Compare To Constant7/1, Compare To Constant6/1
  OV2 Timer/1(out) -> OR/2
  Compare To Constant10/1 -> AND2/1
  Clear Timer1/1(out) -> AND1/1
  OR/1 -> OR4/1
  Clear Timer8/1(out) -> UV2 Timer/1(in)
  AND3/1 -> ac_ok/1, Unit Delay/1  "ac_ok"
  Compare To Constant2/1 -> AND4/1
  Compare To Constant3/1 -> AND5/1
  AND/1 -> Clear Timer1/1(in)
  Compare To Constant/1 -> AND/1
  Compare To Constant1/1 -> AND/2
  AND1/1 -> OR5/1
  OR5/1 -> Assert Timer/1(in)
  to_pu2/1 -> MinMax1/1, MinMax/1
  Clear Timer6/1(out) -> OV1 Timer/1(in)
  OV1 Timer/1(out) -> OR/3
  Clear Timer9/1(out) -> UV3 Timer/1(in)
  UV3 Timer/1(out) -> OR1/3
  MinMax1/1 -> Compare To Constant4/1, Compare To Constant14/1, Compare To Constant5/1, Compare To Constant1/1
  Compare To Constant15/1 -> AND12/1
  OF1 Timer/1(out) -> OR2/3
  Clear Timer12/1(out) -> OF1 Timer/1(in)
  Clear Timer15/1(out) -> UF3 Timer/1(in)
  UF3 Timer/1(out) -> OR3/3
  AND4/1 -> Clear Timer4/1(in)
  Constant/1 -> AND4/2
  AND5/1 -> Clear Timer5/1(in)
  Constant1/1 -> AND5/2
  Compare To Constant13/1 -> AND6/1
  AND6/1 -> Clear Timer6/1(in)
  Constant2/1 -> AND6/2
  Compare To Constant4/1 -> AND7/1
  AND7/1 -> Clear Timer7/1(in)
  Compare To Constant5/1 -> AND8/1
  AND8/1 -> Clear Timer8/1(in)
  Compare To Constant14/1 -> AND9/1
  AND9/1 -> Clear Timer9/1(in)
  Constant3/1 -> AND7/2
  Constant4/1 -> AND8/2
  Constant5/1 -> AND9/2
  AND10/1 -> Clear Timer10/1(in)
  AND11/1 -> Clear Timer11/1(in)
  AND12/1 -> Clear Timer12/1(in)
  Constant6/1 -> AND10/2
  Constant7/1 -> AND11/2
  Constant8/1 -> AND12/2
  Compare To Constant8/1 -> AND13/1
  Constant9/1 -> AND13/2
  Compare To Constant9/1 -> AND14/1
  Constant10/1 -> AND14/2
  AND13/1 -> Clear Timer13/1(in)
  AND14/1 -> Clear Timer14/1(in)
  AND15/1 -> Clear Timer15/1(in)
  Compare To Constant16/1 -> AND15/1
  Constant11/1 -> AND15/2
  OR2/1 -> OR6/1
  OR3/1 -> OR6/2
  OR6/1 -> OR9/2
